simulink model "Projectile_1D"  (R2025b)
settings: Solver=VariableStepAuto  StartTime=0.0  StopTime=15  FixedStep=1e-2  MaxStep=1e-2  RelTol=1e-3
undefined symbols (not defined in the file): g
settings Model: Creator=esmithzb  LastModifiedBy=David
settings SolverCC: EnableFixedStepZeroCrossing=on

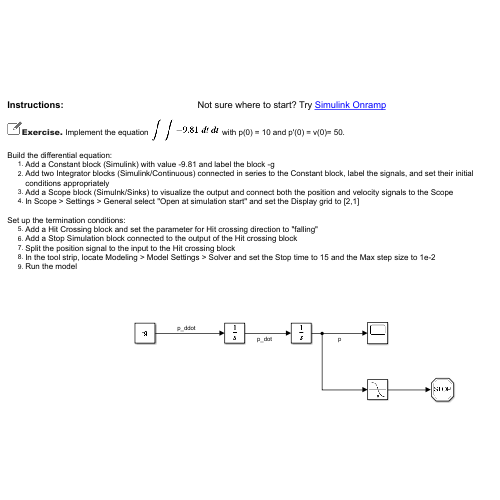
[thumbnail: Simulink's stored preview of the top-level diagram]
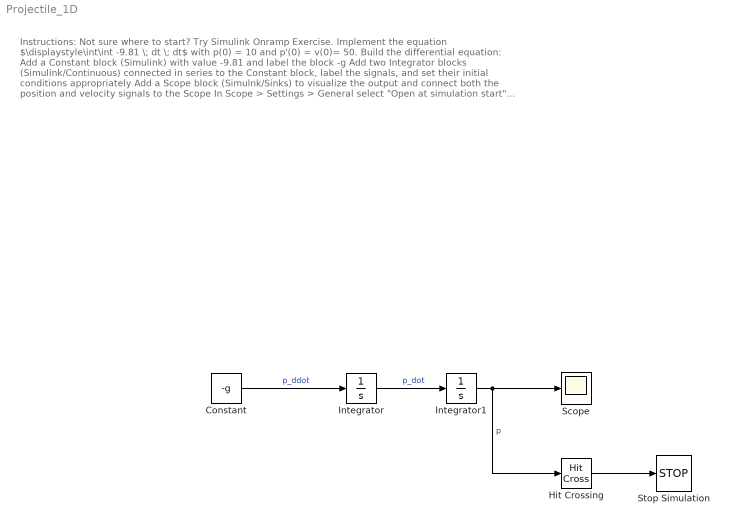
== system Projectile_1D ==
  note: Instructions: Not sure where to start? Try Simulink Onramp
      |
      | Exercise. Implement the equation $\displaystyle\int\int -9.81 \; dt \; dt$ with p(0) = 10 and p'(0) = v(0)= 50.
      |
      | Build the differential equation:
      | Add a Constant block (Simulink) with value -9.81 and label the block -g
      | Add two Integrator blocks (Simulink/Continuous) connected in series to the Constant block, label the signals, and set their initial conditions appropriately
      | Add a Scope block (Simulnk/Sinks) to visualize the output and connect both the position and velocity signals to the Scope
      | In Scope > Settings > General select "Open at simulation start" and set the Display grid to [2,1]
      |
      | Set up the termination conditions:
      | Add a Hit Crossing block and set the parameter for Hit crossing direction to "falling"
      | Add a Stop Simulation block connected to the output of the Hit crossing block
      | Split the position signal to the input to the Hit crossing block
      | In the tool strip, locate Modeling > Model Settings > Solver and set the Stop time to 15 and the Max step size to 1e-2
      | Run the model
  Constant : Constant  Value=-g
  Hit Crossing : HitCross  HitCrossingDirection=falling
  Integrator : Integrator  InitialCondition=60
  Integrator1 : Integrator  InitialCondition=10
  Scope : Scope
      settings: ActiveDisplayYMinimum=-23.70972781250649  ActiveDisplayYMaximum=217.61904531249783
  Stop Simulation : Stop
  wires:
  Integrator/1 -> Integrator1/1  "p_dot"
  Integrator1/1 -> Hit Crossing/1, Scope/1  "p"
  Constant/1 -> Integrator/1  "p_ddot"
  Hit Crossing/1 -> Stop Simulation/1
